simulink model "sf_security"  (R2025b)
settings: Solver=ode5  StartTime=0.0  StopTime=10000  FixedStep=.0001  RelTol=1e-3  AbsTol=1e-6
settings Model: FPTRunName=Active  ExtModeTrigMode=oneshot  ExtModeArmWhenConnect=off  ExtModeAutoUpdateStatusClock=off  Creator=The MathWorks, Inc.  LastModifiedBy=The MathWorks, Inc.
settings SolverCC: AutoScaleAbsTol=off  AlgebraicLoopSolver=TrustRegion  MaxZcPerStep=1.0
settings DataIOCC: SaveFormat=Array  SaveOutput=off  SaveTime=off  ReturnWorkspaceOutputs=off
settings OptimizationCC: BooleanDataType=off  ReuseModelBlockBuffer=off  ExpressionDepthLimit=2147483647.0  InitFltsAndDblsToZero=on  EfficientMapNaN2IntZero=off  LifeSpan=inf  BufferReusableBoundary=off
settings DebuggingCC: SaveWithParameterizedLinksMsg=none  UnderspecifiedInitializationDetection=Classic  MergeDetectMultiDrivingBlocksExec=none  SignalResolutionControl=TryResolveAllWithWarning  MultiTaskDSMMsg=warning  MultiTaskCondExecSysMsg=none  IntegerOverflowMsg=none  FcnCallInpInsideContextMsg=warning  UnconnectedInputMsg=warning  UnconnectedOutputMsg=warning  UnconnectedLineMsg=warning  StateNameClashWarn=warning  SFUnexpectedBacktrackingDiag=warning  SFNoUnconditionalDefaultTransitionDiag=warning  SFExecutionAtInitializationDiag=none  IntegerSaturationMsg=none  ArithmeticOperatorsInVariantConditions=warning
settings HardwareCC: ProdBitPerPointer=32.0  ProdBitPerSizeT=32.0  ProdBitPerPtrDiffT=32.0  ProdLargestAtomicFloat=None  ProdIntDivRoundTo=Undefined  ProdEndianess=Unspecified  ProdWordSize=32.0  ProdHWDeviceType=32-bit Generic  TargetUnknown=on
settings ModelReferenceCC: EnableRefExpFcnMdlSchedulingChecks=on  PropagateSignalLabelsOutOfModel=off
settings SFSimCC: SimUseLocalCustomCode=off  SimParseCustomCode=off  CustomCodeUndefinedFunction=UseInterfaceOnly
settings RTWCC: TemplateMakefile=grt_vc.tmf  RTWUseLocalCustomCode=off  GPUComputeCapability=3.5
settings CodeAppCC: StateflowObjectComments=on
settings GRTTargetCC: TargetFcnLib=ansi_tfl_tmw.mat  TargetLangStandard=C89/C90 (ANSI)  CombineOutputUpdateFcns=off  GRTInterface=on
settings ConfigComp: CovMetricSettings=dcmtr  CovSaveCumulativeToWorkspaceVar=on  CovSaveSingleToWorkspaceVar=on  CovExternalEMLEnable=off  CovSFcnEnable=off

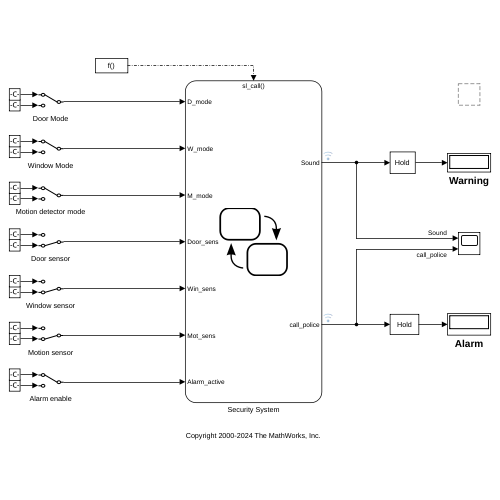
[thumbnail: Simulink's stored preview of the top-level diagram]
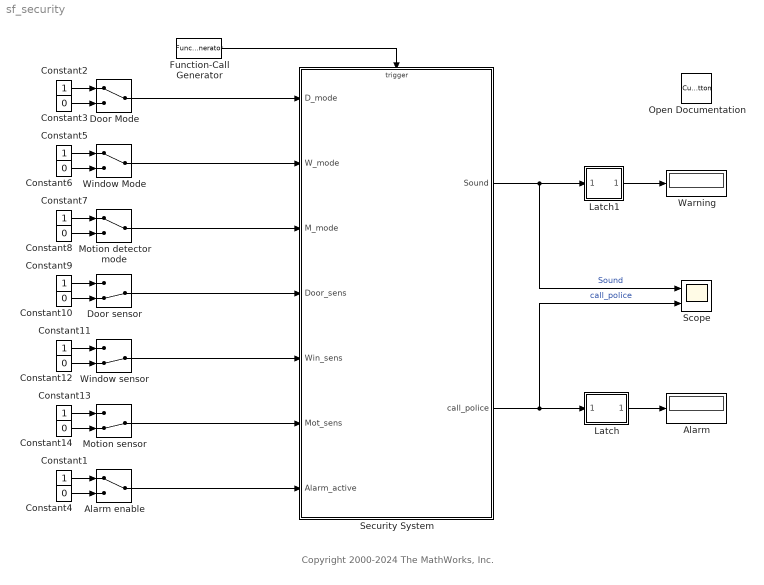
== system sf_security ==
  note: Copyright 2000-2024 The MathWorks, Inc.
  Alarm : Display
  Alarm enable : ManualSwitch
  Constant{1..2,5,7,9,11,13} (7 alike) : Constant  OutDataTypeStr=boolean
  Constant{3..4,6,8,10,12,14} (7 alike) : Constant  Value=0  OutDataTypeStr=boolean
  Door Mode : ManualSwitch
  Door sensor : ManualSwitch  CurrentSetting=0
  Function-Call Generator : FunctionCallGenerator
  Latch : Subsystem
      mask Display: disp('Hold')
  Latch1 : Subsystem
      mask Display: disp('Hold')
  Motion detector mode : ManualSwitch
  Motion sensor : ManualSwitch  CurrentSetting=0
  Open Documentation : CustomCallbackButton  Configuration="{\"components\":[{\"name\":\"BackgroundImageComponent\",\"settings\":{\"image\":{\"size\":[0,0],\"src\":\"default\",\"srcOrientation\":\"Right\"},\"position\":[0,0,1,1]}},{\"name\":\"ButtonStateComponent\",\"settings\":{\"buttonType\":\"momentary\",\"clickFcn\":\"showExample('stateflow\\/EventsGetStartedExample')\",\"onValue\":1,\"position\":[0,0,1,1],\"pressDelay\":\"500\",\"pressFcn\":\"\",\"repeatInterval\":\"0\",\"states\":[{\"horizontalAlignment\":\"center\",\"image\":{\"position\":[0,0,1,1],\"size\":[1,1],\"src\":\"default\",\"srcOrientation\":\"Right\"},\"label\":{\"color\":[0.01176470588,0.01176470588,0.01176470588,1],\"icon\":{\"size\":[0,0],\"src\":\"default\",\"srcOrientation\":\"Right\"},\"iconPlacement\":\"left\",\"opacity\":1,\"show\":true,\"text\":{\"content\":\"?\",\"font\":\"Helvetica\"}},\"labelOffset\":[0,0],\"verticalAlignment\":\"middle\"},{\"horizontalAlignment\":\"center\",\"image\":{\"position\":[0,0,1,1],\"size\":[1,1],\"src\":\"default\",\"srcOrientation\":\"Right\"},\"label\":{\"color\":[0.01176470588,0.01176470588,0.01176470588,1],\"icon\":{\"size\":[0,0],\"src\":\"default\",\"srcOrientation\":\"Right\"},\"iconPlacement\":\"left\",\"opacity\":1,\"show\":true,\"text\":{\"content\":\"?\",\"font\":\"Helvetica\"}},\"labelOffset\":[0,0],\"verticalAlignment\":\"middle\"},{\"horizontalAlignment\":\"center\",\"image\":{\"position\":[0,0,1,1],\"size\":[1,1],\"src\":\"default\",\"srcOrientation\":\"Right\"},\"label\":{\"color\":[0.01176470588,0.01176470588,0.01176470588,1],\"icon\":{\"size\":[0,0],\"src\":\"default\",\"srcOrientation\":\"Right\"},\"iconPlacement\":\"left\",\"opacity\":1,\"show\":true,\"text\":{\"content\":\"?\",\"font\":\"Helvetica\"}},\"labelOffset\":[0,0],\"verticalAlignment\":\"middle\"},{\"horizontalAlignment\":\"center\",\"image\":{\"position\":[0,0,1,1],\"size\":[1,1],\"src\":\"default\",\"srcOrientation\":\"Right\"},\"label\":{\"color\":[0.01176470588,0.01176470588,0.01176470588,1],\"icon\":{\"size\":[0,0],\"src\":\"default\",\"srcOrientation\":\"Right\"},\"iconPlacement\":\"left\",\"opacity\":1,\"show\":true,\"text\":{\"content\":\"?\",\"font\":\"Helvetica\"}},\"labelOffset\":[0,0],\"verticalAlignment\":\"middle\"}]}},{\"name\":\"ForegroundImageComponent\",\"settings\":{\"image\":{\"size\":[0,0],\"src\":\"default\",\"srcOrientation\":\"Right\"},\"isForeground\":1,\"position\":[0,0,1,1]}}],\"settings\":{\"BindingType\":\"standalone\",\"backgroundColor\":[244,244,244,1],\"backgroundOffset\":0,\"backgroundOpacity\":1,\"fixedAspectRatio\":\"off\",\"foregroundColor\":[0.01176470588,0.01176470588,0.01176470588,1],\"migratedFromLegacy\":true,\"useBackgroundColor\":true,\"variant\":\"callback\",\"version\":\"R2024b\"},\"type\":\"Button\"}"  CustomBackgroundColor="{\"color\":[0.9568627451,0.9568627451,0.9568627451],\"show\":true}"
  Scope : Scope  NumInputPorts=2
      settings: TimeSpan=100  ActiveDisplayYMinimum=-0.125  ActiveDisplayYMaximum=1.125  YLabel=Sound  DataLoggingSaveFormat=Structure
  Security System : Stateflow chart  TreatAsAtomicUnit=on
  Warning : Display
  Window Mode : ManualSwitch
  Window sensor : ManualSwitch  CurrentSetting=0
  wires:
  Latch/1(Trigger) -> Alarm/1
  Door Mode/1 -> Security System/1(D_mode)
  Window Mode/1 -> Security System/2(W_mode)
  Motion detector mode/1 -> Security System/3(M_mode)
  Alarm enable/1 -> Security System/7(Alarm_active)
  Motion sensor/1 -> Security System/6(Mot_sens)
  Window sensor/1 -> Security System/5(Win_sens)
  Door sensor/1 -> Security System/4(Door_sens)
  Function-Call Generator/1 -> Security System/Trigger
  Latch1/1(Trigger) -> Warning/1
  Security System/2(call_police) -> Scope/2, Latch/1(Reset)  "call_police"
  Security System/1(Sound) -> Scope/1, Latch1/1(Reset)  "Sound"
  Constant4/1 -> Alarm enable/2
  Constant1/1 -> Alarm enable/1
  Constant3/1 -> Door Mode/2
  Constant2/1 -> Door Mode/1
  Constant6/1 -> Window Mode/2
  Constant5/1 -> Window Mode/1
  Constant8/1 -> Motion detector mode/2
  Constant7/1 -> Motion detector mode/1
  Constant10/1 -> Door sensor/2
  Constant12/1 -> Window sensor/2
  Constant11/1 -> Window sensor/1
  Constant14/1 -> Motion sensor/2
  Constant13/1 -> Motion sensor/1
  Constant9/1 -> Door sensor/1

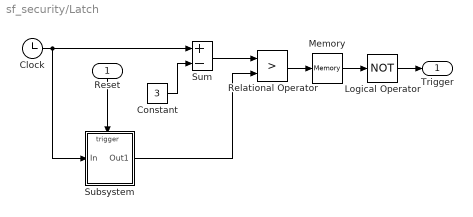
== system sf_security/Latch ==
  Reset : Inport
  Clock : Clock
  Constant : Constant  Value=3
  Logical Operator : Logic  Operator=NOT  Inputs=1
  Memory : Memory  InitialCondition=1
  Relational Operator : RelationalOperator  Operator=>
  Subsystem : Subsystem
  Sum : Sum  Inputs=+-  InputSameDT=on  SaturateOnIntegerOverflow=on  OutDataTypeStr=Inherit: Same as first input
  Trigger : Outport  InitialOutput=0  VectorParamsAs1DForOutWhenUnconnected=off
  wires:
  Clock/1 -> Sum/1, Subsystem/1(In)
  Reset/1 -> Subsystem/Trigger
  Constant/1 -> Sum/2
  Sum/1 -> Relational Operator/1
  Subsystem/1(Out1) -> Relational Operator/2
  Relational Operator/1 -> Memory/1
  Memory/1 -> Logical Operator/1
  Logical Operator/1 -> Trigger/1

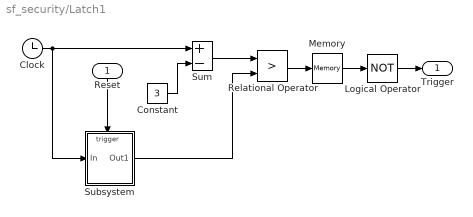
== system sf_security/Latch1 ==
  Reset : Inport
  Clock : Clock
  Constant : Constant  Value=3
  Logical Operator : Logic  Operator=NOT  Inputs=1
  Memory : Memory  InitialCondition=1
  Relational Operator : RelationalOperator  Operator=>
  Subsystem : Subsystem
  Sum : Sum  Inputs=+-  InputSameDT=on  SaturateOnIntegerOverflow=on  OutDataTypeStr=Inherit: Same as first input
  Trigger : Outport  InitialOutput=0  VectorParamsAs1DForOutWhenUnconnected=off
  wires:
  Logical Operator/1 -> Trigger/1
  Memory/1 -> Logical Operator/1
  Relational Operator/1 -> Memory/1
  Subsystem/1(Out1) -> Relational Operator/2
  Sum/1 -> Relational Operator/1
  Constant/1 -> Sum/2
  Reset/1 -> Subsystem/Trigger
  Clock/1 -> Subsystem/1(In), Sum/1

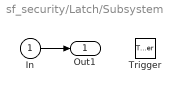
== system sf_security/Latch/Subsystem ==
  In : Inport
  Trigger : TriggerPort  TriggerType=either  VariantControl=Variant
  Out1 : Outport  InitialOutput=-10  VectorParamsAs1DForOutWhenUnconnected=off
  wires:
  In/1 -> Out1/1

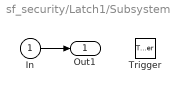
== system sf_security/Latch1/Subsystem ==
  In : Inport
  Trigger : TriggerPort  TriggerType=either  VariantControl=Variant
  Out1 : Outport  InitialOutput=-10  VectorParamsAs1DForOutWhenUnconnected=off
  wires:
  In/1 -> Out1/1

== stateflow chart sf_security/Security System ==
  state Motion [parallel]
    settings: executionOrder=2  description=This state models the modes of a motion detector sensor and implements logic to respond when that sensor is producing a signal.
    state Active
      state Debouncing
      state Idle
      Debouncing -> Debouncing [order 1] : after(delay,sl_call)
          | [in(Alarm.On.Idle)]
          | {send(Alert,Alarm)}
      Debouncing -> Motion.Active.Idle [order 2] : [~Mot_sens]
      Motion.Active.Idle -> Debouncing : [Mot_sens]
    state Disabled
    (default) -> Motion.Active.Idle
      settings: description=On the first sample call the motion sensor mode is set to active, in the idle substate.
    Motion.Disabled -> Motion.Active.Idle : [M_mode==1]
    Motion.Active -> Motion.Disabled : [M_mode==0]
  state Door [parallel]
    settings: executionOrder=1  description=This state models the modes of a door sensor and implements logic to respond when that sensor is producing a signal.
    state Disabled
    state Active
      Door.Active -> (junction 46) [order 1] : [Door_sens && ...
          |  in(Alarm.On.Idle)]
          | {send(Alert,Alarm)}
    Door.Disabled -> Door.Active : [D_mode==1]
    (default) -> Door.Active
      settings: description=On the first sample call the door mode is set to active.
    Door.Active -> Door.Disabled [order 1] : [D_mode==0]
  state Win [parallel]
    settings: executionOrder=3  description=This state models the modes of a window sensor and implements logic to respond when that sensor is producing a signal.
    state Disabled
    state Active
      Win.Active -> (junction 43) [order 1] : [Win_sens && ...
          | in(Alarm.On.Idle)]
          | {send(Alert,Alarm)}
    Win.Disabled -> Win.Active : [W_mode==1]
    (default) -> Win.Active
      settings: description=On the first sample call the window mode is set to active.
    Win.Active -> Win.Disabled [order 1] : [W_mode==0]
  state Alarm [parallel]
    settings: executionOrder=4
    state On
      state Pending
        entry:
        send(Sound)
      state Idle
      (default) -> Alarm.On.Idle
      Alarm.On.Idle -> Pending : Alert
      Pending -> Alarm.On.Idle : after(4*delay,sl_call)
          | {send(call_police)}
    state Off
    (default) -> On
      settings: description=On the first sample call the Alarm is set to active.
    On -> Off : [Alarm_active==0]
    Off -> On : [Alarm_active==1]
  data: D_mode input boolean; W_mode input boolean; M_mode input boolean; Door_sens input boolean; Win_sens input boolean; Mot_sens input boolean; Alarm_active input boolean; delay constant double =20
  events: Sound output EITHER_EDGE_EVENT; call_police output EITHER_EDGE_EVENT; Alert local EITHER_EDGE_EVENT; sl_call input FUNCTION_CALL_EVENT
